simulink model "furuta_double_inverted_pendulum_model"  (R2025a)
settings: Solver=ode4  StartTime=0.0  StopTime=inf  FixedStep=0.001  RelTol=1e-3
InitFcn:
  | addpath('functions');
model workspace (MATLAB code in the model file):
  | L_arm = 0.2;
  | I_arm = 0.01;
  | L_1 = 1;
  | lcom_1 = 0.6;
  | I_1 = 0.02;
  | m_1 = 1;
  | L_2 = 0.8;
  | lcom_2 = 0.4;
  | I_2 = 0.02;
  | m_2 = 0.8;
  | 
  | init_cond = [pi/2; 0; 0.01; 0; 0; 0];
settings Model: Creator=Esther  LastModifiedBy=Esther

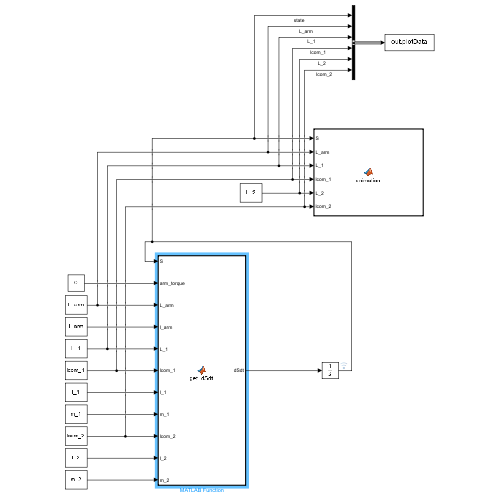
[thumbnail: Simulink's stored preview of the top-level diagram]
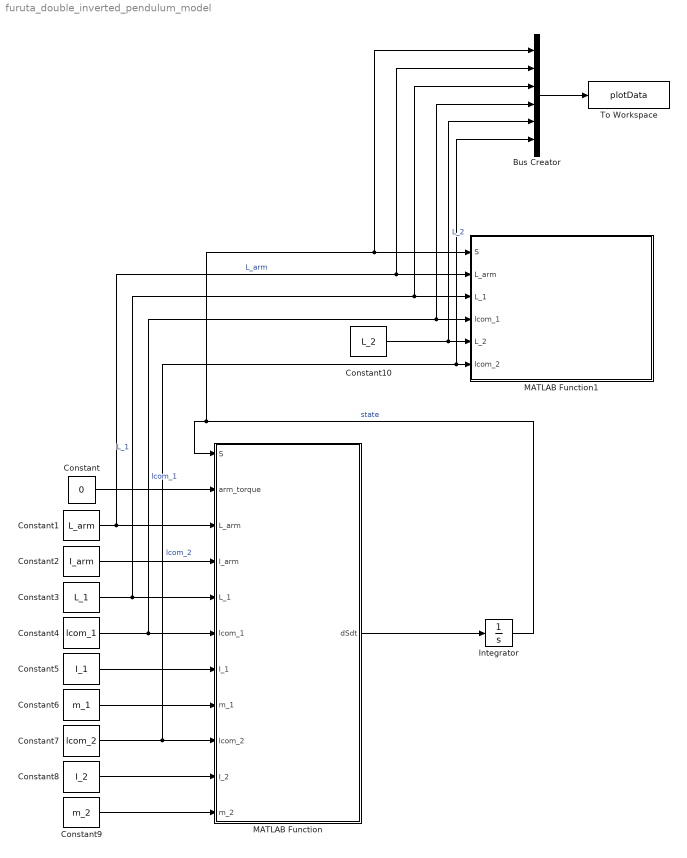
== system furuta_double_inverted_pendulum_model ==
  Bus Creator : BusCreator  Inputs=6
  Constant : Constant  Value=0
  Constant1 : Constant  Value=L_arm
  Constant10 : Constant  Value=L_2
  Constant2 : Constant  Value=I_arm
  Constant3 : Constant  Value=L_1
  Constant4 : Constant  Value=lcom_1
  Constant5 : Constant  Value=I_1
  Constant6 : Constant  Value=m_1
  Constant7 : Constant  Value=lcom_2
  Constant8 : Constant  Value=I_2
  Constant9 : Constant  Value=m_2
  Integrator : Integrator  InitialCondition=init_cond
  MATLAB Function : MATLAB Function  TreatAsAtomicUnit=on
  MATLAB Function1 : MATLAB Function  TreatAsAtomicUnit=on
  To Workspace : ToWorkspace  VariableName=plotData  SaveFormat=Timeseries  SampleTime=-1
  wires:
  MATLAB Function/1(dSdt) -> Integrator/1
  Constant/1 -> MATLAB Function/2(arm_torque)
  Constant1/1 -> MATLAB Function/3(L_arm), Bus Creator/2, MATLAB Function1/2(L_arm)  "L_arm"
  Constant2/1 -> MATLAB Function/4(I_arm)
  Constant3/1 -> MATLAB Function/5(L_1), Bus Creator/3, MATLAB Function1/3(L_1)  "L_1"
  Constant4/1 -> Bus Creator/4, MATLAB Function1/4(lcom_1), MATLAB Function/6(lcom_1)  "lcom_1"
  Constant5/1 -> MATLAB Function/7(I_1)
  Constant6/1 -> MATLAB Function/8(m_1)
  Constant7/1 -> Bus Creator/6, MATLAB Function1/6(lcom_2), MATLAB Function/9(lcom_2)  "lcom_2"
  Constant8/1 -> MATLAB Function/10(I_2)
  Constant9/1 -> MATLAB Function/11(m_2)
  Constant10/1 -> MATLAB Function1/5(L_2), Bus Creator/5  "L_2"
  Bus Creator/1 -> To Workspace/1
  Integrator/1 -> Bus Creator/1, MATLAB Function1/1(S), MATLAB Function/1(S)  "state"

== matlab function furuta_double_inverted_pendulum_model/MATLAB Function1 ==
  settings: updateMethod=DISCRETE
  data: S input; L_arm input; L_1 input; lcom_1 input; L_2 input; lcom_2 input
function animation(S, L_arm, L_1, lcom_1, L_2, lcom_2)
    update_ratio = 100;
    realtime_animation_double(S, L_arm, L_1, lcom_1, L_2, lcom_2, update_ratio)
end

== matlab function furuta_double_inverted_pendulum_model/MATLAB Function ==
  data: dSdt output size=6; S input size=6; arm_torque input size=1; L_arm input size=1; I_arm input size=1; L_1 input size=1; lcom_1 input size=1; I_1 input size=1; m_1 input size=1; lcom_2 input size=1; I_2 input size=1; m_2 input size=1
function dSdt = get_dSdt(S, arm_torque, L_arm, I_arm, L_1, lcom_1, I_1, m_1, lcom_2, I_2, m_2)
    t = 0;
    g = 9.81;

    phys_param_double = [L_arm, I_arm, L_1, lcom_1, I_1, m_1, lcom_2, I_2, m_2, g];
    fric_arm = [0.018, 0.018, 100];
    fric_1 = [0.0001, 0.0001, 100];
    fric_2 = [0.0001, 0.0001, 100];

    dSdt = furuta_double_state_derivative(t, S, arm_torque, phys_param_double, fric_arm, fric_1, fric_2);

end
